simulink model "lab_otu_observer"  (R2022a)
settings: Solver=VariableStepAuto  StartTime=0.0  StopTime=10.0  RelTol=1e-3
undefined symbols (not defined in the file): A, B, C, D, F, L, T
libraries: simulink x2
settings Model: Creator=salgi  LastModifiedBy=salgi

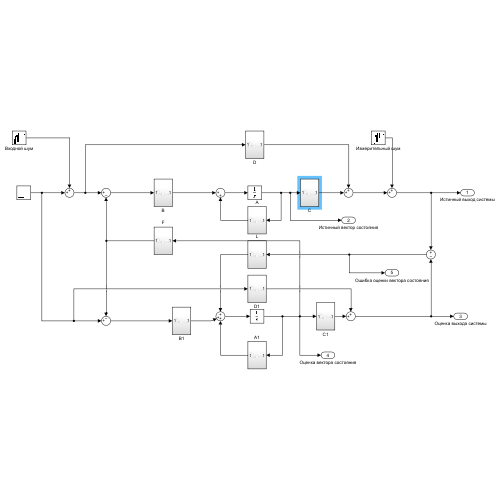
[thumbnail: Simulink's stored preview of the top-level diagram]
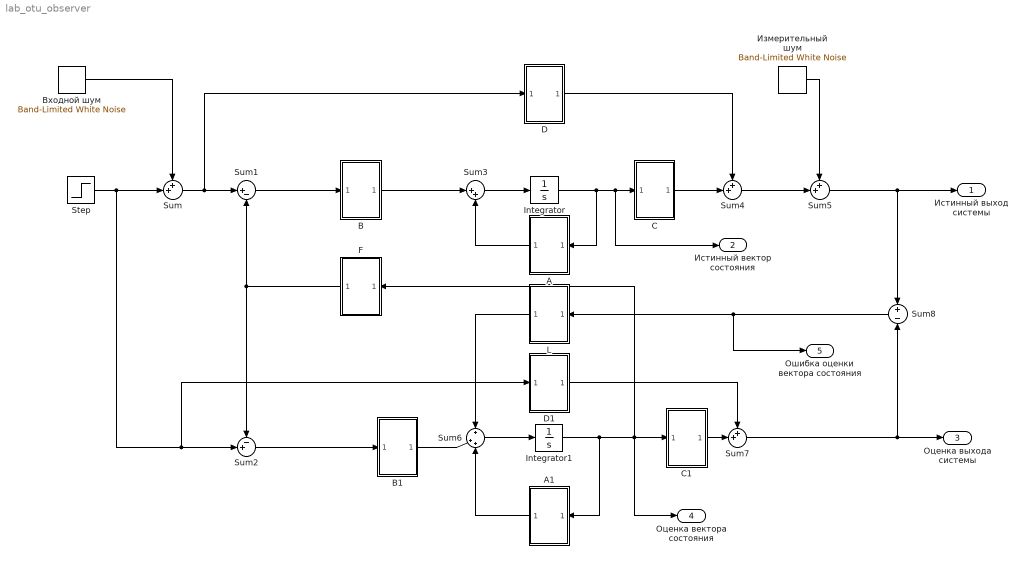
== system lab_otu_observer ==
  A : Subsystem
  A1 : Subsystem
  B : Subsystem
  B1 : Subsystem
  C : Subsystem
  C1 : Subsystem
  D : Subsystem
  D1 : Subsystem
  F : Subsystem
  Integrator : Integrator
  Integrator1 : Integrator
  L : Subsystem
  Step : Step  Time=1.0  Before=0.0  After=1.0  SampleTime=T  VectorParams1D=off
  Sum{,4..5,7} (4 alike) : Sum  Inputs=++|
  Sum1 : Sum  Inputs=|+-
  Sum2 : Sum  Inputs=-+|
  Sum3 : Sum  Inputs=|++
  Sum6 : Sum  Inputs=+|++
  Sum8 : Sum  Inputs=+-
  Входной шум : simulink/Sources/Band-Limited White Noise  Cov=cov_Input  Ts=T  seed=[23341]
  Измерительный шум : simulink/Sources/Band-Limited White Noise  Cov=cov_Output  Ts=T  seed=[23341]
  Истинный выход системы : Outport
  Истинный вектор состояния : Outport  Port=2
  Оценка выхода системы : Outport  Port=3
  Оценка вектора состояния : Outport  Port=4
  Ошибка оценки вектора состояния : Outport  Port=5
  wires:
  Step/1 -> D1/1(In1), Sum2/2, Sum/2
  Входной шум/1 -> Sum/1
  Sum/1 -> D/1(In1), Sum1/1
  Sum3/1 -> Integrator/1
  Измерительный шум/1 -> Sum5/1
  Sum2/1 -> B1/1(In1)
  B1/1(Out3) -> Sum6/2
  Sum6/1 -> Integrator1/1
  Integrator/1 -> A/1(In1), Истинный вектор состояния/1, C/1(In1)
  C/1(Out3) -> Sum4/2
  A/1(Out3) -> Sum3/2
  B/1(Out3) -> Sum3/1
  Sum1/1 -> B/1(In1)
  C1/1(Out3) -> Sum7/2
  Integrator1/1 -> A1/1(In1), F/1(In1), Оценка вектора состояния/1, C1/1(In1)
  F/1(Out3) -> Sum1/2, Sum2/1
  L/1(Out3) -> Sum6/1
  A1/1(Out3) -> Sum6/3
  D1/1(Out3) -> Sum7/1
  Sum7/1 -> Оценка выхода системы/1, Sum8/2
  Sum5/1 -> Истинный выход системы/1, Sum8/1
  Sum8/1 -> Ошибка оценки вектора состояния/1, L/1(In1)
  Sum4/1 -> Sum5/2
  D/1(Out3) -> Sum4/1

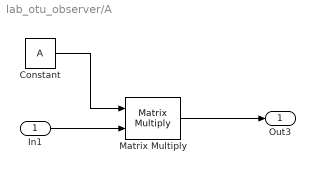
== system lab_otu_observer/A ==
  In1 : Inport
  Constant : Constant  Value=A  VectorParams1D=off
  Matrix Multiply : Product  Multiplication=Matrix(*)
  Out3 : Outport
  wires:
  In1/1 -> Matrix Multiply/2
  Constant/1 -> Matrix Multiply/1
  Matrix Multiply/1 -> Out3/1

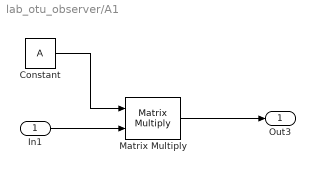
== system lab_otu_observer/A1 ==
  In1 : Inport
  Constant : Constant  Value=A  VectorParams1D=off
  Matrix Multiply : Product  Multiplication=Matrix(*)
  Out3 : Outport
  wires:
  In1/1 -> Matrix Multiply/2
  Constant/1 -> Matrix Multiply/1
  Matrix Multiply/1 -> Out3/1

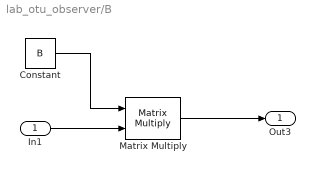
== system lab_otu_observer/B ==
  In1 : Inport
  Constant : Constant  Value=B  VectorParams1D=off
  Matrix Multiply : Product  Multiplication=Matrix(*)
  Out3 : Outport
  wires:
  In1/1 -> Matrix Multiply/2
  Constant/1 -> Matrix Multiply/1
  Matrix Multiply/1 -> Out3/1

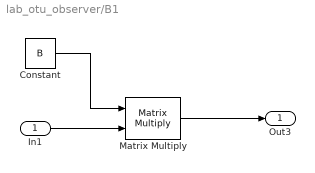
== system lab_otu_observer/B1 ==
  In1 : Inport
  Constant : Constant  Value=B  VectorParams1D=off
  Matrix Multiply : Product  Multiplication=Matrix(*)
  Out3 : Outport
  wires:
  In1/1 -> Matrix Multiply/2
  Constant/1 -> Matrix Multiply/1
  Matrix Multiply/1 -> Out3/1

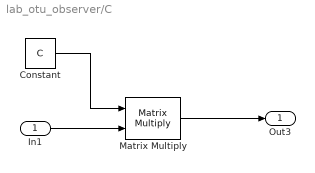
== system lab_otu_observer/C ==
  In1 : Inport
  Constant : Constant  Value=C  VectorParams1D=off
  Matrix Multiply : Product  Multiplication=Matrix(*)
  Out3 : Outport
  wires:
  In1/1 -> Matrix Multiply/2
  Constant/1 -> Matrix Multiply/1
  Matrix Multiply/1 -> Out3/1

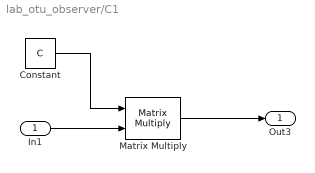
== system lab_otu_observer/C1 ==
  In1 : Inport
  Constant : Constant  Value=C  VectorParams1D=off
  Matrix Multiply : Product  Multiplication=Matrix(*)
  Out3 : Outport
  wires:
  In1/1 -> Matrix Multiply/2
  Constant/1 -> Matrix Multiply/1
  Matrix Multiply/1 -> Out3/1

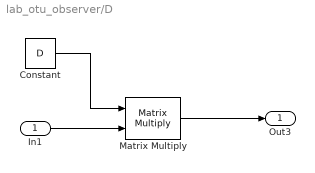
== system lab_otu_observer/D ==
  In1 : Inport
  Constant : Constant  Value=D  VectorParams1D=off
  Matrix Multiply : Product  Multiplication=Matrix(*)
  Out3 : Outport
  wires:
  In1/1 -> Matrix Multiply/2
  Constant/1 -> Matrix Multiply/1
  Matrix Multiply/1 -> Out3/1

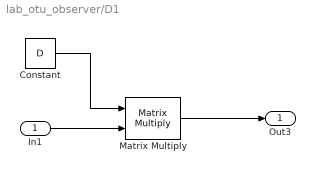
== system lab_otu_observer/D1 ==
  In1 : Inport
  Constant : Constant  Value=D  VectorParams1D=off
  Matrix Multiply : Product  Multiplication=Matrix(*)
  Out3 : Outport
  wires:
  In1/1 -> Matrix Multiply/2
  Constant/1 -> Matrix Multiply/1
  Matrix Multiply/1 -> Out3/1

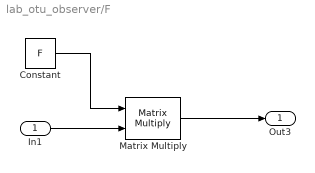
== system lab_otu_observer/F ==
  In1 : Inport
  Constant : Constant  Value=F  VectorParams1D=off
  Matrix Multiply : Product  Multiplication=Matrix(*)
  Out3 : Outport
  wires:
  In1/1 -> Matrix Multiply/2
  Constant/1 -> Matrix Multiply/1
  Matrix Multiply/1 -> Out3/1

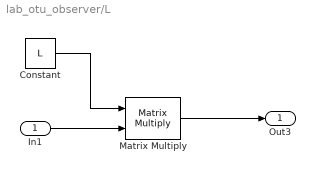
== system lab_otu_observer/L ==
  In1 : Inport
  Constant : Constant  Value=L  VectorParams1D=off
  Matrix Multiply : Product  Multiplication=Matrix(*)
  Out3 : Outport
  wires:
  In1/1 -> Matrix Multiply/2
  Constant/1 -> Matrix Multiply/1
  Matrix Multiply/1 -> Out3/1
